simulink model "Hybrid_OpAmp_Full"
settings: Solver=ode23t  StopTime=0.002  RelTol=1e-5  AbsTol=1e-6
settings Model: Creator=Senior Analog IC & SET Device Design Engineer  LastModifiedBy=Antigravity MATLAB Automation

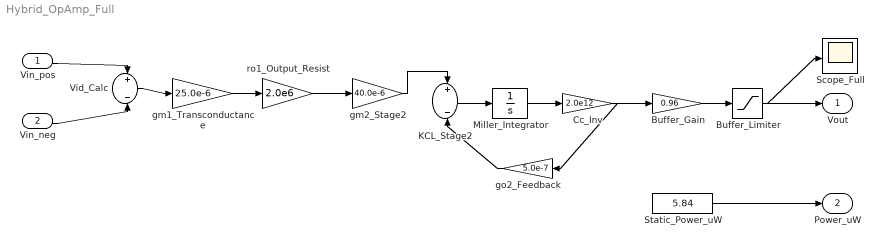
== system Hybrid_OpAmp_Full ==
  Vin_pos : Inport  Port=1
  Vin_neg : Inport  Port=2
  Vid_Calc : Sum  Inputs=+-
  gm1_Transconductance : Gain  Gain=25.0e-6
  ro1_Output_Resist : Gain  Gain=2.0e6
  gm2_Stage2 : Gain  Gain=40.0e-6
  KCL_Stage2 : Sum  Inputs=+-
  Miller_Integrator : Integrator  InitialCondition=0.4  LimitOutput=on  UpperSaturationLimit=0.75  LowerSaturationLimit=0.05
  Cc_Inv : Gain  Gain=2.0e12
  go2_Feedback : Gain  Gain=5.0e-7  Orientation=left
  Buffer_Gain : Gain  Gain=0.96
  Buffer_Limiter : Saturate  UpperLimit=0.75  LowerLimit=0.05
  Static_Power_uW : Constant  Value=5.84
  Vout : Outport  Port=1
  Power_uW : Outport  Port=2
  Scope_Full : Scope
  wires:
  Vin_pos/1 -> Vid_Calc/1
  Vin_neg/1 -> Vid_Calc/2
  Vid_Calc/1 -> gm1_Transconductance/1
  gm1_Transconductance/1 -> ro1_Output_Resist/1
  ro1_Output_Resist/1 -> gm2_Stage2/1
  gm2_Stage2/1 -> KCL_Stage2/1
  KCL_Stage2/1 -> Miller_Integrator/1
  Miller_Integrator/1 -> Cc_Inv/1
  Cc_Inv/1 -> Buffer_Gain/1
  Cc_Inv/1 -> go2_Feedback/1
  go2_Feedback/1 -> KCL_Stage2/2
  Buffer_Gain/1 -> Buffer_Limiter/1
  Buffer_Limiter/1 -> Vout/1
  Buffer_Limiter/1 -> Scope_Full/1
  Static_Power_uW/1 -> Power_uW/1
